simulink model "MMC_Per_arm_outer_v5_G2_case2_clip_delay1p4_aligned"  (R2024a)
settings: Solver=FixedStepDiscrete  StartTime=0.0  StopTime=2  FixedStep=Ts  RelTol=1e-3
PreLoadFcn:
  | % ---- MMC_Inner4 workspace parameters (control gains live inside the MATLAB Function blocks) ----
  | % ---------------- Converter ----------------
  | VDC     = 800;                  % DC-link voltage (V)  -> Vdc_pos / Vdc_neg = VDC/2
  | N       = 8;                    % submodules per arm
  | C       = 2.2e-3;               % submodule capacitance (F)  -> HB_xx blocks
  | vo      = 100;                  % nominal = initial capacitor voltage (V) = VDC/N  -> HB_xx, Vc_nom
  | W_nom   = 0.5*C*N*vo^2;         % nominal arm energy (J) -> initial condition of the Comm delay blocks
  | Larm    = 5e-3;                 % arm inductance (H)
  | Rarm    = 0.5;                  % arm resistance (ohm)
  | 
  | % ---------------- Grid and PCC filter ----------------
  | f       = 50;                   % grid frequency (Hz)
  | Vg_rms  = 230;                  % grid RMS voltage (V)
  | Vg_pk   = Vg_rms*sqrt(2);       % grid peak voltage (V) -> AC Voltage Source
  | Lg      = 2e-3;                 % line inductance (H)
  | Rg      = 0.1;                  % line resistance (ohm)
  | Cf      = 10e-6;                % AC filter capacitance (F)
  | Rf      = 10;                   % AC filter damping resistance (ohm)
  | 
  | % ---------------- Power set-points ----------------
  | Pstar   = 1500;                 % active-power set-point (W)
  | Qstar   = 0;                    % reactive-power set-point (var)
  | 
  | % ---------------- Timing ----------------
  | fsw     = 1250;                 % carrier frequency per submodule (Hz) -> N*fsw = 10 kHz per arm
  | Ts      = 1e-5;                 % simulation step = submodule-layer step (s)
  | Ts_ctrl = 1e-4;                 % arm-leader control step (s)
  | % ---------------- Test schedule: P* staircase and PCC load (added in _tests) ----------------
  | P_base   = 1500;                % staircase base = first level (W)
  | dP_step  = 250;                 % staircase step (W): 1500 -> 1750 -> 2000 -> 2250 -> 2500
  | t_step   = [0.6 1.0 1.4 1.8];   % step instants (s), 0.4 s hold at each level
  | t_back   = 2.2;                 % return to P_base (s) before the load test
  | P_load1  = 1000;                % PCC load 1 (W at 230 V rms)
  | P_load2  = 1000;                % PCC load 2 (W at 230 V rms)
  | R_load1  = Vg_rms^2/P_load1;    % 52.9 ohm
  | R_load2  = Vg_rms^2/P_load2;    % 52.9 ohm
  | t_load1  = 2.4;                 % Breaker load 1: closes at 2.4 s (stays closed)
  | t_load2  = [2.7 3.0];           % Breaker load 2: closes at 2.7 s, opens at 3.0 s
  | % ---- CASE: initial imbalance HB_u3 = 110 V, HB_u6 = 90 V, P* fixed 1500 W, no PCC load, 2 s
  | % ---- DERIVED: case2_clip_delay1p4_aligned: case 2 clip + time-aligned delay 140 samples (1.4 ms) -- eq. (6) test below the bound
  | % ---- DERIVED: case2_clip: same as case 2 + correction bounded to |k_v*err| <= 0.1 in hb_sm_local_ctrl (16 charts)
  | % P_SLEW = 5000 W/s, I_max = 17 A, P_max = 2500 W are set INSIDE mmc_outer_ctrl (both arm leaders)
  | t_load1  = 10;  t_load2 = [10 11];   % PCC load test disabled in this case (beyond StopTime)
  | Vc0_u3   = 110;                 % initial capacitor voltage of HB_u3 (V)
  | Vc0_u6   = 90;                  % initial capacitor voltage of HB_u6 (V)
InitFcn:
  | % ---- MMC_Inner4 workspace parameters (control gains live inside the MATLAB Function blocks) ----
  | % ---------------- Converter ----------------
  | VDC     = 800;                  % DC-link voltage (V)  -> Vdc_pos / Vdc_neg = VDC/2
  | N       = 8;                    % submodules per arm
  | C       = 2.2e-3;               % submodule capacitance (F)  -> HB_xx blocks
  | vo      = 100;                  % nominal = initial capacitor voltage (V) = VDC/N  -> HB_xx, Vc_nom
  | W_nom   = 0.5*C*N*vo^2;         % nominal arm energy (J) -> initial condition of the Comm delay blocks
  | Larm    = 5e-3;                 % arm inductance (H)
  | Rarm    = 0.5;                  % arm resistance (ohm)
  | 
  | % ---------------- Grid and PCC filter ----------------
  | f       = 50;                   % grid frequency (Hz)
  | Vg_rms  = 230;                  % grid RMS voltage (V)
  | Vg_pk   = Vg_rms*sqrt(2);       % grid peak voltage (V) -> AC Voltage Source
  | Lg      = 2e-3;                 % line inductance (H)
  | Rg      = 0.1;                  % line resistance (ohm)
  | Cf      = 10e-6;                % AC filter capacitance (F)
  | Rf      = 10;                   % AC filter damping resistance (ohm)
  | 
  | % ---------------- Power set-points ----------------
  | Pstar   = 1500;                 % active-power set-point (W)
  | Qstar   = 0;                    % reactive-power set-point (var)
  | 
  | % ---------------- Timing ----------------
  | fsw     = 1250;                 % carrier frequency per submodule (Hz) -> N*fsw = 10 kHz per arm
  | Ts      = 1e-5;                 % simulation step = submodule-layer step (s)
  | Ts_ctrl = 1e-4;                 % arm-leader control step (s)
  | % ---------------- Test schedule: P* staircase and PCC load (added in _tests) ----------------
  | P_base   = 1500;                % staircase base = first level (W)
  | dP_step  = 250;                 % staircase step (W): 1500 -> 1750 -> 2000 -> 2250 -> 2500
  | t_step   = [0.6 1.0 1.4 1.8];   % step instants (s), 0.4 s hold at each level
  | t_back   = 2.2;                 % return to P_base (s) before the load test
  | P_load1  = 1000;                % PCC load 1 (W at 230 V rms)
  | P_load2  = 1000;                % PCC load 2 (W at 230 V rms)
  | R_load1  = Vg_rms^2/P_load1;    % 52.9 ohm
  | R_load2  = Vg_rms^2/P_load2;    % 52.9 ohm
  | t_load1  = 2.4;                 % Breaker load 1: closes at 2.4 s (stays closed)
  | t_load2  = [2.7 3.0];           % Breaker load 2: closes at 2.7 s, opens at 3.0 s
  | % ---- CASE: initial imbalance HB_u3 = 110 V, HB_u6 = 90 V, P* fixed 1500 W, no PCC load, 2 s
  | % ---- DERIVED: case2_clip_delay1p4_aligned: case 2 clip + time-aligned delay 140 samples (1.4 ms) -- eq. (6) test below the bound
  | % ---- DERIVED: case2_clip: same as case 2 + correction bounded to |k_v*err| <= 0.1 in hb_sm_local_ctrl (16 charts)
  | % P_SLEW = 5000 W/s, I_max = 17 A, P_max = 2500 W are set INSIDE mmc_outer_ctrl (both arm leaders)
  | t_load1  = 10;  t_load2 = [10 11];   % PCC load test disabled in this case (beyond StopTime)
  | Vc0_u3   = 110;                 % initial capacitor voltage of HB_u3 (V)
  | Vc0_u6   = 90;                  % initial capacitor voltage of HB_u6 (V)
libraries: spsHalfBridgeMMCLib x16, spsSeriesRLCBranchLib x6, spsCurrentMeasurementLib x5, spsBreakerLib x2, spsGroundLib x2, spsDCVoltageSourceLib x2, spsACVoltageSourceLib x1, spspowerguiLib x1, spsVoltageMeasurementLib x1
(part 1 of 6)
settings Model: Creator=Dell  LastModifiedBy=Dell
settings SolverCC: AutoInsertRateTranBlk=on

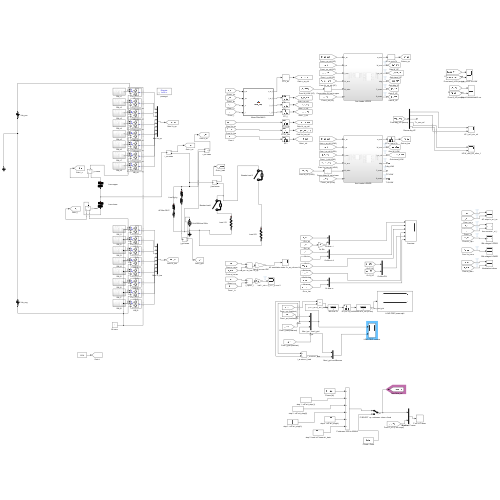
[thumbnail: Simulink's stored preview of the top-level diagram]
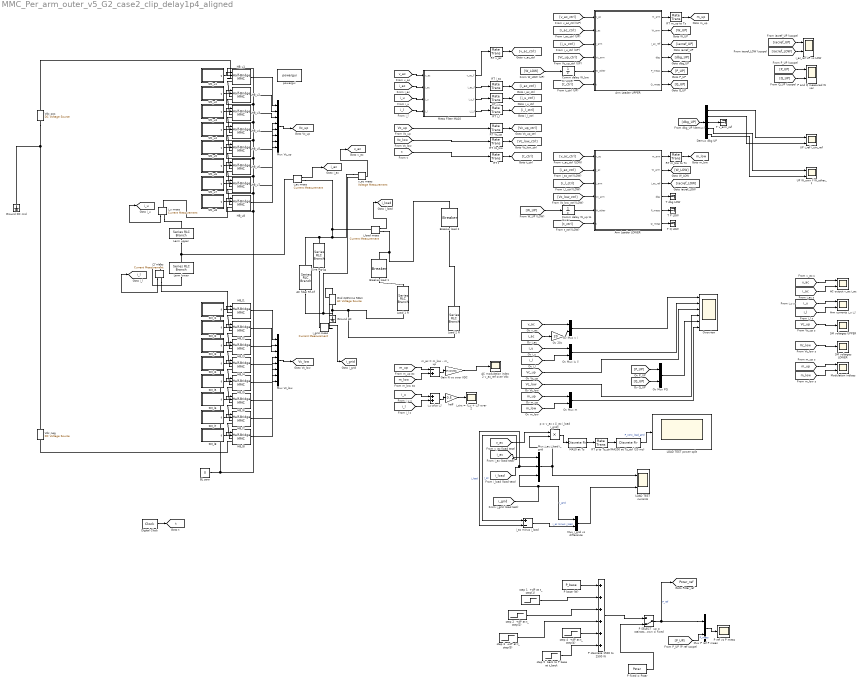
== system MMC_Per_arm_outer_v5_G2_case2_clip_delay1p4_aligned ==
  AC filter Rf-Cf : spsSeriesRLCBranchLib/Series RLC Branch  LConnTagsString=__new0  RConnTagsString=__new0  BranchType=RC  Resistance=Rf  Inductance=1e-3  SetiL0=off  InitialCurrent=0  Capacitance=Cf  Setx0=off  InitialVoltage=0  Measurements=None
  AC modulation index 2 v_ac_ref over Vdc : Scope
  AC output v_ac i_ac : Scope  NumInputPorts=2
  Arm Leader LOWER : Subsystem
  Arm Leader UPPER : Subsystem
  Arm currents i_u i_l : Scope  NumInputPorts=2
  BL zero : Constant  Value=0
  Breaker load 1 : spsBreakerLib/Breaker  InitialState=0  SwitchingTimes=t_load1  External=off  BreakerResistance=0.01  SnubberResistance=1e6  SnubberCapacitance=inf  Measurements=None  MoreParameters=on  NoBreakLoop=off
  Breaker load 2 : spsBreakerLib/Breaker  InitialState=0  SwitchingTimes=t_load2  External=off  BreakerResistance=0.01  SnubberResistance=1e6  SnubberCapacitance=inf  Measurements=None  MoreParameters=on  NoBreakLoop=off
  Comm delay W_low to upper : UnitDelay  InitialCondition=W_nom  SampleTime=Ts_ctrl  HasFrameUpgradeWarning=on
  Comm delay W_up to lower : UnitDelay  InitialCondition=W_nom  SampleTime=Ts_ctrl  HasFrameUpgradeWarning=on
  Demux dbg UP : Demux  Outputs=5
  Digital Clock : DigitalClock  SampleTime=Ts
  Gain N vo over VDC : Gain  Gain=N*vo/VDC
  Grid 230Vrms 50Hz : spsACVoltageSourceLib/AC Voltage Source  Amplitude=Vg_pk  Phase=0  Frequency=f  SampleTime=0  Measurements=None  BusType=swing  Pref=10e3  Qref=0  Qmin=-inf  Qmax=+inf
  Ground AC : spsGroundLib/Ground  LConnTagsString=a
  Ground DC mid : spsGroundLib/Ground  LConnTagsString=a
  HB_l{1..8} (8 alike) : spsHalfBridgeMMCLib/Half-Bridge MMC  ModelType=Switching devices  n=1  C=C  Vc_Initial=vo  Ron=1e-3  Rs=1e6  Cs=inf  Ron_Diode=1e-3  Rs_Diode=1e6  Cs_Diode=inf  Vf_Diode=1e-3  Rs_CurrentSource=inf  Ts=Ts
  HB_u{1..2,4..5,7..8} (6 alike) : spsHalfBridgeMMCLib/Half-Bridge MMC  ModelType=Switching devices  n=1  C=C  Vc_Initial=vo  Ron=1e-3  Rs=1e6  Cs=inf  Ron_Diode=1e-3  Rs_Diode=1e6  Cs_Diode=inf  Vf_Diode=1e-3  Rs_CurrentSource=inf  Ts=Ts
  HB_u3 : spsHalfBridgeMMCLib/Half-Bridge MMC  ModelType=Switching devices  n=1  C=C  Vc_Initial=Vc0_u3  Ron=1e-3  Rs=1e6  Cs=inf  Ron_Diode=1e-3  Rs_Diode=1e6  Cs_Diode=inf  Vf_Diode=1e-3  Rs_CurrentSource=inf  Ts=Ts
  HB_u6 : spsHalfBridgeMMCLib/Half-Bridge MMC  ModelType=Switching devices  n=1  C=C  Vc_Initial=Vc0_u6  Ron=1e-3  Rs=1e6  Cs=inf  Ron_Diode=1e-3  Rs_Diode=1e6  Cs_Diode=inf  Vf_Diode=1e-3  Rs_CurrentSource=inf  Ts=Ts
  LOAD TEST currents : Scope  NumInputPorts=2
  LOAD TEST power split : Scope
  Larm lower : spsSeriesRLCBranchLib/Series RLC Branch  LConnTagsString=__new0  RConnTagsString=__new0  BranchType=RL  Resistance=Rarm  Inductance=Larm  SetiL0=off  InitialCurrent=0  Capacitance=1e-6  Setx0=off  InitialVoltage=0  Measurements=None
  Larm upper : spsSeriesRLCBranchLib/Series RLC Branch  LConnTagsString=__new0  RConnTagsString=__new0  BranchType=RL  Resistance=Rarm  Inductance=Larm  SetiL0=off  InitialCurrent=0  Capacitance=1e-6  Setx0=off  InitialVoltage=0  Measurements=None
  Line Rg-Lg : spsSeriesRLCBranchLib/Series RLC Branch  LConnTagsString=__new0  RConnTagsString=__new0  BranchType=RL  Resistance=Rg  Inductance=Lg  SetiL0=off  InitialCurrent=0  Capacitance=1e-6  Setx0=off  InitialVoltage=0  Measurements=None
  Load 1 R : spsSeriesRLCBranchLib/Series RLC Branch  LConnTagsString=__new0  RConnTagsString=__new0  BranchType=R  Resistance=R_load1  Inductance=1e-3  SetiL0=off  InitialCurrent=0  Capacitance=1e-6  Setx0=off  InitialVoltage=0  Measurements=None
  Load 2 R : spsSeriesRLCBranchLib/Series RLC Branch  LConnTagsString=__new0  RConnTagsString=__new0  BranchType=R  Resistance=R_load2  Inductance=1e-3  SetiL0=off  InitialCurrent=0  Capacitance=1e-6  Setx0=off  InitialVoltage=0  Measurements=None
  MA10 at Ts : DiscreteFir  Coefficients=ones(1,10)/10  SampleTime=Ts
  MA200 at Ts_ctrl (20 ms) : DiscreteFir  Coefficients=ones(1,200)/200  SampleTime=Ts_ctrl
  Meas Filter MA10 : MATLAB Function  TreatAsAtomicUnit=on
  Modulation indices : Scope  NumInputPorts=2
  Mux P ref P meas : Mux  Inputs=2
  Mux Vc_low : Mux  Inputs=8
  Mux Vc_up : Mux  Inputs=8
  Mux i_ac i_load i_grid : Mux  Inputs=3
  Mux i_grid vs difference : Mux  Inputs=2
  Ov 20x : Gain  Gain=20
  Ov Mux PQ : Mux  Inputs=2
  Ov Mux iu il : Mux  Inputs=2
  Ov Mux m : Mux  Inputs=2
  Ov Mux v i : Mux  Inputs=2
  Overview : Scope  NumInputPorts=6
  P SELECT  up = staircase  down = fixed : ManualSwitch  sw=0
  P and Q measured W var : Scope  NumInputPorts=2
  P base (W) : Constant  Value=P_base
  P fixed = Pstar : Constant  Value=Pstar
  P ref vs P meas : Scope
  P staircase 1500 to 2500 W : Sum  Inputs=++++++
  RT Vc_low : RateTransition  OutPortSampleTime=Ts_ctrl
  RT Vc_up : RateTransition  OutPortSampleTime=Ts_ctrl
  RT i_ac : RateTransition  OutPortSampleTime=Ts_ctrl
  RT i_l : RateTransition  OutPortSampleTime=Ts_ctrl
  RT i_u : RateTransition  OutPortSampleTime=Ts_ctrl
  RT m_low to Ts : RateTransition  Deterministic=off  OutPortSampleTime=Ts
  RT m_up to Ts : RateTransition  Deterministic=off  OutPortSampleTime=Ts
  RT p to Ts_ctrl : RateTransition  OutPortSampleTime=Ts_ctrl
  RT t : RateTransition  OutPortSampleTime=Ts_ctrl
  RT v_ac : RateTransition  OutPortSampleTime=Ts_ctrl
  SM voltages LOWER : Scope
  SM voltages UPPER : Scope
  SM_l1 : Subsystem
  SM_l2 : Subsystem
  SM_l3 : Subsystem
  SM_l4 : Subsystem
  SM_l5 : Subsystem
  SM_l6 : Subsystem
  SM_l7 : Subsystem
  SM_l8 : Subsystem
  SM_u1 : Subsystem
  SM_u2 : Subsystem
  SM_u3 : Subsystem
  SM_u4 : Subsystem
  SM_u5 : Subsystem
  SM_u6 : Subsystem
  SM_u7 : Subsystem
  SM_u8 : Subsystem
  T P LOW : Terminator
  T Q LOW : Terminator
  T dbg LOW : Terminator
  T v_arm_ref : Terminator
  UP W_own_f W_other_f : Scope  NumInputPorts=2
  UP i_ref i_circ_ref : Scope  NumInputPorts=2
  Vdc_neg : spsDCVoltageSourceLib/DC Voltage Source  Amplitude=VDC/2  Measurements=None
  Vdc_pos : spsDCVoltageSourceLib/DC Voltage Source  Amplitude=VDC/2  Measurements=None
  half : Gain  Gain=0.5
  i_ac meas : spsCurrentMeasurementLib/Current Measurement  PhasorSimulation=off  OutputType=Complex  PSBequivalent=0
  i_ac minus i_load : Sum  Inputs=+-
  i_ac_ref UP vs LOW : Scope  NumInputPorts=2
  i_circ = (i_u + i_l) over 2 : Scope
  i_grid meas : spsCurrentMeasurementLib/Current Measurement  PhasorSimulation=off  OutputType=Complex  PSBequivalent=0
  i_l meas : spsCurrentMeasurementLib/Current Measurement  PhasorSimulation=off  OutputType=Complex  PSBequivalent=0
  i_load meas : spsCurrentMeasurementLib/Current Measurement  PhasorSimulation=off  OutputType=Complex  PSBequivalent=0
  i_u meas : spsCurrentMeasurementLib/Current Measurement  PhasorSimulation=off  OutputType=Complex  PSBequivalent=0
  i_u plus i_l : Sum
  m_ac = m_low - m_up : Sum  Inputs=-+
  p = v_ac x [i_ac i_load i_grid] : Product
  powergui : spspowerguiLib/powergui  Priority=1  SimulationMode=Discrete  SampleTime=Ts  frequency=50  Iterations=50  frequencyindice=50  Pbase=100e6  ErrMax=1e-4  UnitsV=kV  UnitsW=MW  buscounter=0  FunctionMessages=off  echomessages=off  EnableUseOfTLC=off  CurrentSourceSwitches=off  DisableSnubberDevices=off  DisableRonSwitches=off  DisableVfSwitches=off  DisplayEquations=off  AutomaticDiscreteSolvers=off  SolverType=Tustin/Backward Euler (TBE)  Interpol=off  ExternalGateDelay=off  methode=off  Ts=100  x0status=blocks  SPID=on  SwTol=0  HookPort=off  NonlinearTolerance=1e-4  nMaxIteration=100  ContinueOnMaxIteration=off  RestoreLinks=warning  ResistiveCurrentMeasurement=off  Frange=[0:2:500]  Ylog=off  Xlog=on  ShowGrid=off  save=off  variable=ZData  structure=0  ZoomFFT=off  StartTime=0.0  cycles=1  DisplayStyle=1  fundamental=50  FreqAxis=off  MaxFrequency=1000  frequencyindicesteady=1  RmsSteady=1  display=off
  step 1  +dP at t_step(1) : Step  Time=t_step(1)  After=dP_step  SampleTime=Ts_ctrl
  step 2  +dP at t_step(2) : Step  Time=t_step(2)  After=dP_step  SampleTime=Ts_ctrl
  step 3  +dP at t_step(3) : Step  Time=t_step(3)  After=dP_step  SampleTime=Ts_ctrl
  step 4  +dP at t_step(4) : Step  Time=t_step(4)  After=dP_step  SampleTime=Ts_ctrl
  step 5  back to P base at t_back : Step  Time=t_back  After=-4*dP_step  SampleTime=Ts_ctrl
  v_ac meas : spsVoltageMeasurementLib/Voltage Measurement  PhasorSimulation=off  OutputType=Complex  PSBequivalent=0
  tag scope: Pstar_ref=global, Vc_low=global, Vc_up=global, i_ac=global, i_grid=global, i_l=global, i_load=global, i_u=global, m_low=global, m_up=global, t=global, v_ac=global
  wires:
  v_ac meas/1 -> [v_ac]
  i_ac meas/1 -> [i_ac]
  i_u meas/1 -> [i_u]
  i_l meas/1 -> [i_l]
  BL zero/1 -> HB_u1/2, HB_u2/2, HB_u3/2, HB_u4/2, HB_u5/2, HB_u6/2, HB_u7/2, HB_u8/2, HB_l1/2, HB_l2/2, HB_l3/2, HB_l4/2, HB_l5/2, HB_l6/2, HB_l7/2, HB_l8/2
  HB_u1/1 -> Mux Vc_up/1
  HB_l1/1 -> Mux Vc_low/1
  HB_u2/1 -> Mux Vc_up/2
  HB_l2/1 -> Mux Vc_low/2
  HB_u3/1 -> Mux Vc_up/3
  HB_l3/1 -> Mux Vc_low/3
  HB_u4/1 -> Mux Vc_up/4
  HB_l4/1 -> Mux Vc_low/4
  HB_u5/1 -> Mux Vc_up/5
  HB_l5/1 -> Mux Vc_low/5
  HB_u6/1 -> Mux Vc_up/6
  HB_l6/1 -> Mux Vc_low/6
  HB_u7/1 -> Mux Vc_up/7
  HB_l7/1 -> Mux Vc_low/7
  HB_u8/1 -> Mux Vc_up/8
  HB_l8/1 -> Mux Vc_low/8
  Mux Vc_up/1 -> [Vc_up]
  Mux Vc_low/1 -> [Vc_low]
  Digital Clock/1 -> [t]
  SM_u1/1(g) -> HB_u1/1
  SM_l1/1(g) -> HB_l1/1
  SM_u2/1(g) -> HB_u2/1
  SM_l2/1(g) -> HB_l2/1
  SM_u3/1(g) -> HB_u3/1
  SM_l3/1(g) -> HB_l3/1
  SM_u4/1(g) -> HB_u4/1
  SM_l4/1(g) -> HB_l4/1
  SM_u5/1(g) -> HB_u5/1
  SM_l5/1(g) -> HB_l5/1
  SM_u6/1(g) -> HB_u6/1
  SM_l6/1(g) -> HB_l6/1
  SM_u7/1(g) -> HB_u7/1
  SM_l7/1(g) -> HB_l7/1
  SM_u8/1(g) -> HB_u8/1
  SM_l8/1(g) -> HB_l8/1
  [v_ac] -> Meas Filter MA10/1(v_ac)
  [i_ac] -> Meas Filter MA10/2(i_ac)
  [i_u] -> Meas Filter MA10/3(i_u)
  [i_l] -> Meas Filter MA10/4(i_l)
  Meas Filter MA10/1(v_ac_f) -> RT v_ac/1
  Meas Filter MA10/2(i_ac_f) -> RT i_ac/1
  Meas Filter MA10/3(i_u_f) -> RT i_u/1
  Meas Filter MA10/4(i_l_f) -> RT i_l/1
  [Vc_up] -> RT Vc_up/1
  [Vc_low] -> RT Vc_low/1
  [t] -> RT t/1
  [v_ac] -> AC output v_ac i_ac/1
  [i_ac] -> AC output v_ac i_ac/2
  [i_u] -> Arm currents i_u i_l/1
  [i_l] -> Arm currents i_u i_l/2
  [Vc_up] -> SM voltages UPPER/1
  [Vc_low] -> SM voltages LOWER/1
  [m_up] -> Modulation indices/1
  [m_low] -> Modulation indices/2
  [m_up] -> m_ac = m_low - m_up/1
  [m_low] -> m_ac = m_low - m_up/2
  m_ac = m_low - m_up/1 -> Gain N vo over VDC/1
  Gain N vo over VDC/1 -> AC modulation index 2 v_ac_ref over Vdc/1
  [i_u] -> i_u plus i_l/1
  [i_l] -> i_u plus i_l/2
  i_u plus i_l/1 -> half/1
  half/1 -> i_circ = (i_u + i_l) over 2/1
  Demux dbg UP/1 -> UP i_ref i_circ_ref/1
  Demux dbg UP/2 -> UP i_ref i_circ_ref/2
  Demux dbg UP/3 -> T v_arm_ref/1
  Demux dbg UP/4 -> UP W_own_f W_other_f/1
  Demux dbg UP/5 -> UP W_own_f W_other_f/2
  [v_ac] -> Ov Mux v i/1
  [i_ac] -> Ov 20x/1
  Ov 20x/1 -> Ov Mux v i/2
  [i_u] -> Ov Mux iu il/1
  [i_l] -> Ov Mux iu il/2
  [m_up] -> Ov Mux m/1
  [m_low] -> Ov Mux m/2
  Ov Mux v i/1 -> Overview/1
  Ov Mux iu il/1 -> Overview/2
  [Vc_up] -> Overview/3
  [Vc_low] -> Overview/4
  Ov Mux PQ/1 -> Overview/5
  Ov Mux m/1 -> Overview/6
  RT v_ac/1 -> [v_ac_ctrl]
  RT i_ac/1 -> [i_ac_ctrl]
  RT i_u/1 -> [i_u_ctrl]
  RT i_l/1 -> [i_l_ctrl]
  RT Vc_up/1 -> [Vc_up_ctrl]
  RT Vc_low/1 -> [Vc_low_ctrl]
  RT t/1 -> [t_ctrl]
  [v_ac_ctrl] -> Arm Leader UPPER/1(v_ac)
  [i_ac_ctrl] -> Arm Leader UPPER/2(i_ac)
  [i_u_ctrl] -> Arm Leader UPPER/3(i_arm)
  [Vc_up_ctrl] -> Arm Leader UPPER/4(Vc_arm)
  [W_LOW] -> Comm delay W_low to upper/1
  Comm delay W_low to upper/1 -> Arm Leader UPPER/5(W_other)
  [t_ctrl] -> Arm Leader UPPER/6(t)
  [v_ac_ctrl] -> Arm Leader LOWER/1(v_ac)
  [i_ac_ctrl] -> Arm Leader LOWER/2(i_ac)
  [i_l_ctrl] -> Arm Leader LOWER/3(i_arm)
  [Vc_low_ctrl] -> Arm Leader LOWER/4(Vc_arm)
  [W_UP] -> Comm delay W_up to lower/1
  Comm delay W_up to lower/1 -> Arm Leader LOWER/5(W_other)
  [t_ctrl] -> Arm Leader LOWER/6(t)
  Arm Leader UPPER/1(m_arm) -> RT m_up to Ts/1
  RT m_up to Ts/1 -> [m_up]
  Arm Leader UPPER/2(W_arm) -> [W_UP]
  Arm Leader UPPER/3(i_ac_ref) -> [iacref_UP]
  Arm Leader UPPER/4(dbg) -> [dbg_UP]
  Arm Leader UPPER/5(P_meas) -> [P_UP]
  Arm Leader UPPER/6(Q_meas) -> [Q_UP]
  Arm Leader LOWER/1(m_arm) -> RT m_low to Ts/1
  RT m_low to Ts/1 -> [m_low]
  Arm Leader LOWER/2(W_arm) -> [W_LOW]
  Arm Leader LOWER/3(i_ac_ref) -> [iacref_LOW]
  Arm Leader LOWER/4(dbg) -> T dbg LOW/1
  Arm Leader LOWER/5(P_meas) -> T P LOW/1
  Arm Leader LOWER/6(Q_meas) -> T Q LOW/1
  [iacref_UP] -> i_ac_ref UP vs LOW/1
  [iacref_LOW] -> i_ac_ref UP vs LOW/2
  [P_UP] -> P and Q measured W var/1
  [Q_UP] -> P and Q measured W var/2
  [dbg_UP] -> Demux dbg UP/1
  [P_UP] -> Ov Mux PQ/1
  [Q_UP] -> Ov Mux PQ/2
  P base (W)/1 -> P staircase 1500 to 2500 W/1
  step 1  +dP at t_step(1)/1 -> P staircase 1500 to 2500 W/2
  step 2  +dP at t_step(2)/1 -> P staircase 1500 to 2500 W/3
  step 3  +dP at t_step(3)/1 -> P staircase 1500 to 2500 W/4
  step 4  +dP at t_step(4)/1 -> P staircase 1500 to 2500 W/5
  step 5  back to P base at t_back/1 -> P staircase 1500 to 2500 W/6
  P staircase 1500 to 2500 W/1 -> P SELECT  up = staircase  down = fixed/1
  P fixed = Pstar/1 -> P SELECT  up = staircase  down = fixed/2
  P SELECT  up = staircase  down = fixed/1 -> [Pstar_ref], Mux P ref P meas/1  "P_ref"
  [P_UP] -> Mux P ref P meas/2  "P_meas"
  Mux P ref P meas/1 -> P ref vs P meas/1
  i_load meas/1 -> [i_load]
  i_grid meas/1 -> [i_grid]
  [i_ac] -> Mux i_ac i_load i_grid/1, i_ac minus i_load/1  "i_ac"
  [i_load] -> Mux i_ac i_load i_grid/2, i_ac minus i_load/2  "i_load"
  [i_grid] -> Mux i_ac i_load i_grid/3, Mux i_grid vs difference/1  "i_grid"
  i_ac minus i_load/1 -> Mux i_grid vs difference/2  "i_ac minus i_load"
  Mux i_ac i_load i_grid/1 -> p = v_ac x [i_ac i_load i_grid]/2, LOAD TEST currents/1
  Mux i_grid vs difference/1 -> LOAD TEST currents/2
  [v_ac] -> p = v_ac x [i_ac i_load i_grid]/1
  p = v_ac x [i_ac i_load i_grid]/1 -> MA10 at Ts/1
  MA10 at Ts/1 -> RT p to Ts_ctrl/1
  RT p to Ts_ctrl/1 -> MA200 at Ts_ctrl (20 ms)/1
  MA200 at Ts_ctrl (20 ms)/1 -> LOAD TEST power split/1  "P_conv_load_grid"
  connections:
  HB_u1/LConn1 -- Vdc_pos/RConn1
  Vdc_pos/LConn1 -- Ground DC mid/LConn1 -- Vdc_neg/RConn1
  HB_u1/LConn2 -- HB_u2/LConn1
  HB_l1/LConn2 -- HB_l2/LConn1
  HB_u2/LConn2 -- HB_u3/LConn1
  HB_l2/LConn2 -- HB_l3/LConn1
  HB_u3/LConn2 -- HB_u4/LConn1
  HB_l3/LConn2 -- HB_l4/LConn1
  HB_u4/LConn2 -- HB_u5/LConn1
  HB_l4/LConn2 -- HB_l5/LConn1
  HB_u5/LConn2 -- HB_u6/LConn1
  HB_l5/LConn2 -- HB_l6/LConn1
  HB_u6/LConn2 -- HB_u7/LConn1
  HB_l6/LConn2 -- HB_l7/LConn1
  HB_u7/LConn2 -- HB_u8/LConn1
  HB_l7/LConn2 -- HB_l8/LConn1
  HB_u8/LConn2 -- i_u meas/LConn1
  i_u meas/RConn1 -- Larm upper/LConn1
  Larm upper/RConn1 -- i_ac meas/LConn1 -- Larm lower/LConn1
  Larm lower/RConn1 -- i_l meas/LConn1
  i_l meas/RConn1 -- HB_l1/LConn1
  HB_l8/LConn2 -- Vdc_neg/LConn1
  v_ac meas/LConn1 -- Line Rg-Lg/LConn1 -- AC filter Rf-Cf/LConn1 -- i_ac meas/RConn1 -- i_load meas/LConn1
  Line Rg-Lg/RConn1 -- i_grid meas/LConn1
  Grid 230Vrms 50Hz/LConn1 -- Load 1 R/RConn1 -- Load 2 R/RConn1 -- AC filter Rf-Cf/RConn1 -- v_ac meas/LConn2 -- Ground AC/LConn1
  i_load meas/RConn1 -- Breaker load 2/LConn1 -- Breaker load 1/LConn1
  Breaker load 1/RConn1 -- Load 1 R/LConn1
  Breaker load 2/RConn1 -- Load 2 R/LConn1
  i_grid meas/RConn1 -- Grid 230Vrms 50Hz/RConn1

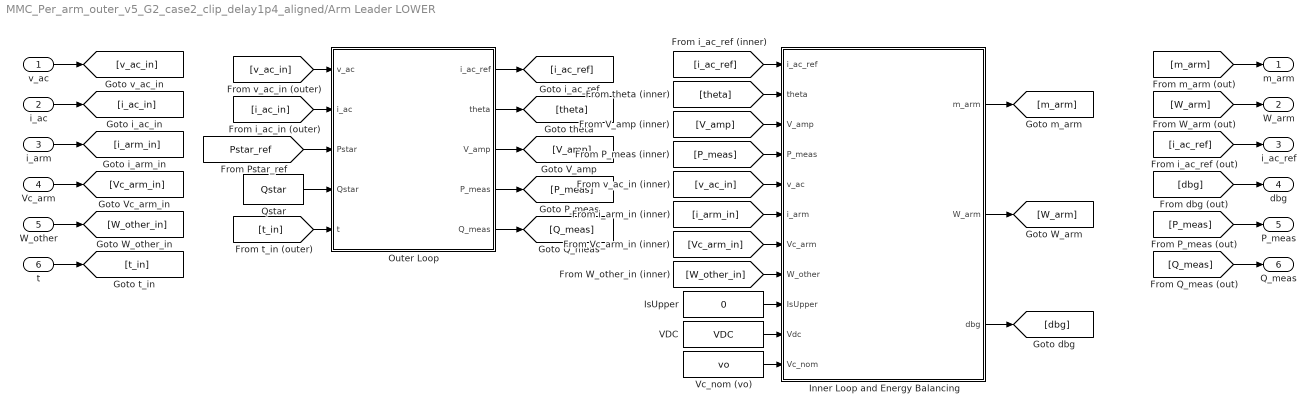
== system MMC_Per_arm_outer_v5_G2_case2_clip_delay1p4_aligned/Arm Leader LOWER ==
  v_ac : Inport
  i_ac : Inport  Port=2
  i_arm : Inport  Port=3
  Vc_arm : Inport  Port=4
  W_other : Inport  Port=5
  t : Inport  Port=6
  Inner Loop and Energy Balancing : Subsystem
  IsUpper : Constant  Value=0
  Outer Loop : MATLAB Function  TreatAsAtomicUnit=on
  Qstar : Constant  Value=Qstar
  VDC : Constant  Value=VDC
  Vc_nom (vo) : Constant  Value=vo
  m_arm : Outport
  W_arm : Outport  Port=2
  i_ac_ref : Outport  Port=3
  dbg : Outport  Port=4
  P_meas : Outport  Port=5
  Q_meas : Outport  Port=6
  wires:
  v_ac/1 -> [v_ac_in]
  i_ac/1 -> [i_ac_in]
  i_arm/1 -> [i_arm_in]
  Vc_arm/1 -> [Vc_arm_in]
  W_other/1 -> [W_other_in]
  t/1 -> [t_in]
  [v_ac_in] -> Outer Loop/1(v_ac)
  [i_ac_in] -> Outer Loop/2(i_ac)
  [Pstar_ref] -> Outer Loop/3(Pstar)
  Qstar/1 -> Outer Loop/4(Qstar)
  [t_in] -> Outer Loop/5(t)
  Outer Loop/1(i_ac_ref) -> [i_ac_ref]
  Outer Loop/2(theta) -> [theta]
  Outer Loop/3(V_amp) -> [V_amp]
  Outer Loop/4(P_meas) -> [P_meas]
  Outer Loop/5(Q_meas) -> [Q_meas]
  [i_ac_ref] -> Inner Loop and Energy Balancing/1(i_ac_ref)
  [theta] -> Inner Loop and Energy Balancing/2(theta)
  [V_amp] -> Inner Loop and Energy Balancing/3(V_amp)
  [P_meas] -> Inner Loop and Energy Balancing/4(P_meas)
  [v_ac_in] -> Inner Loop and Energy Balancing/5(v_ac)
  [i_arm_in] -> Inner Loop and Energy Balancing/6(i_arm)
  [Vc_arm_in] -> Inner Loop and Energy Balancing/7(Vc_arm)
  [W_other_in] -> Inner Loop and Energy Balancing/8(W_other)
  IsUpper/1 -> Inner Loop and Energy Balancing/9(IsUpper)
  VDC/1 -> Inner Loop and Energy Balancing/10(Vdc)
  Vc_nom (vo)/1 -> Inner Loop and Energy Balancing/11(Vc_nom)
  Inner Loop and Energy Balancing/1(m_arm) -> [m_arm]
  Inner Loop and Energy Balancing/2(W_arm) -> [W_arm]
  Inner Loop and Energy Balancing/3(dbg) -> [dbg]
  [m_arm] -> m_arm/1
  [W_arm] -> W_arm/1
  [i_ac_ref] -> i_ac_ref/1
  [dbg] -> dbg/1
  [P_meas] -> P_meas/1
  [Q_meas] -> Q_meas/1

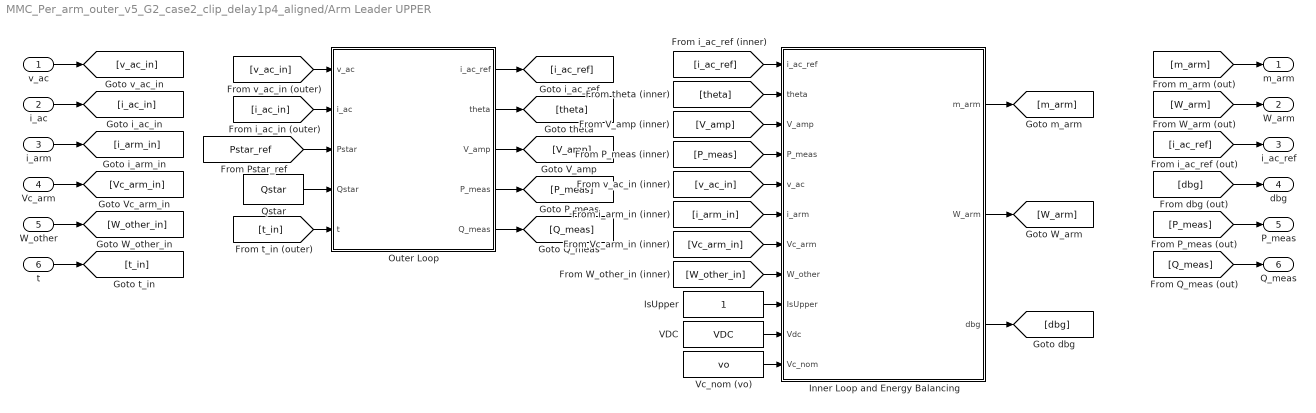
== system MMC_Per_arm_outer_v5_G2_case2_clip_delay1p4_aligned/Arm Leader UPPER ==
  v_ac : Inport
  i_ac : Inport  Port=2
  i_arm : Inport  Port=3
  Vc_arm : Inport  Port=4
  W_other : Inport  Port=5
  t : Inport  Port=6
  Inner Loop and Energy Balancing : Subsystem
  IsUpper : Constant
  Outer Loop : MATLAB Function  TreatAsAtomicUnit=on
  Qstar : Constant  Value=Qstar
  VDC : Constant  Value=VDC
  Vc_nom (vo) : Constant  Value=vo
  m_arm : Outport
  W_arm : Outport  Port=2
  i_ac_ref : Outport  Port=3
  dbg : Outport  Port=4
  P_meas : Outport  Port=5
  Q_meas : Outport  Port=6
  wires:
  v_ac/1 -> [v_ac_in]
  i_ac/1 -> [i_ac_in]
  i_arm/1 -> [i_arm_in]
  Vc_arm/1 -> [Vc_arm_in]
  W_other/1 -> [W_other_in]
  t/1 -> [t_in]
  [v_ac_in] -> Outer Loop/1(v_ac)
  [i_ac_in] -> Outer Loop/2(i_ac)
  [Pstar_ref] -> Outer Loop/3(Pstar)
  Qstar/1 -> Outer Loop/4(Qstar)
  [t_in] -> Outer Loop/5(t)
  Outer Loop/1(i_ac_ref) -> [i_ac_ref]
  Outer Loop/2(theta) -> [theta]
  Outer Loop/3(V_amp) -> [V_amp]
  Outer Loop/4(P_meas) -> [P_meas]
  Outer Loop/5(Q_meas) -> [Q_meas]
  [i_ac_ref] -> Inner Loop and Energy Balancing/1(i_ac_ref)
  [theta] -> Inner Loop and Energy Balancing/2(theta)
  [V_amp] -> Inner Loop and Energy Balancing/3(V_amp)
  [P_meas] -> Inner Loop and Energy Balancing/4(P_meas)
  [v_ac_in] -> Inner Loop and Energy Balancing/5(v_ac)
  [i_arm_in] -> Inner Loop and Energy Balancing/6(i_arm)
  [Vc_arm_in] -> Inner Loop and Energy Balancing/7(Vc_arm)
  [W_other_in] -> Inner Loop and Energy Balancing/8(W_other)
  IsUpper/1 -> Inner Loop and Energy Balancing/9(IsUpper)
  VDC/1 -> Inner Loop and Energy Balancing/10(Vdc)
  Vc_nom (vo)/1 -> Inner Loop and Energy Balancing/11(Vc_nom)
  Inner Loop and Energy Balancing/1(m_arm) -> [m_arm]
  Inner Loop and Energy Balancing/2(W_arm) -> [W_arm]
  Inner Loop and Energy Balancing/3(dbg) -> [dbg]
  [m_arm] -> m_arm/1
  [W_arm] -> W_arm/1
  [i_ac_ref] -> i_ac_ref/1
  [dbg] -> dbg/1
  [P_meas] -> P_meas/1
  [Q_meas] -> Q_meas/1

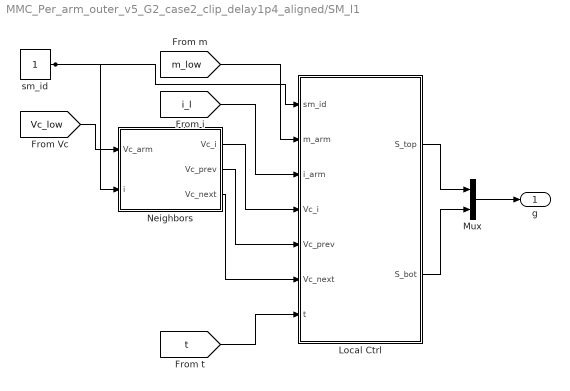
== system MMC_Per_arm_outer_v5_G2_case2_clip_delay1p4_aligned/SM_l1 ==
  Local Ctrl : MATLAB Function  TreatAsAtomicUnit=on
  Mux : Mux  Inputs=2
  Neighbors : MATLAB Function  TreatAsAtomicUnit=on
  sm_id : Constant
  g : Outport
  wires:
  [Vc_low] -> Neighbors/1(Vc_arm)
  sm_id/1 -> Neighbors/2(i), Local Ctrl/1(sm_id)
  [m_low] -> Local Ctrl/2(m_arm)
  [i_l] -> Local Ctrl/3(i_arm)
  Neighbors/1(Vc_i) -> Local Ctrl/4(Vc_i)
  Neighbors/2(Vc_prev) -> Local Ctrl/5(Vc_prev)
  Neighbors/3(Vc_next) -> Local Ctrl/6(Vc_next)
  [t] -> Local Ctrl/7(t)
  Local Ctrl/1(S_top) -> Mux/1
  Local Ctrl/2(S_bot) -> Mux/2
  Mux/1 -> g/1

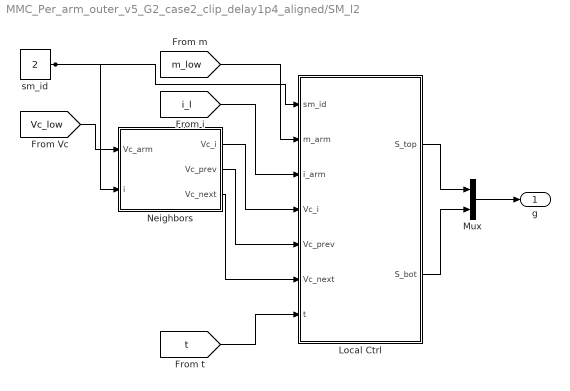
== system MMC_Per_arm_outer_v5_G2_case2_clip_delay1p4_aligned/SM_l2 ==
  Local Ctrl : MATLAB Function  TreatAsAtomicUnit=on
  Mux : Mux  Inputs=2
  Neighbors : MATLAB Function  TreatAsAtomicUnit=on
  sm_id : Constant  Value=2
  g : Outport
  wires:
  [Vc_low] -> Neighbors/1(Vc_arm)
  sm_id/1 -> Neighbors/2(i), Local Ctrl/1(sm_id)
  [m_low] -> Local Ctrl/2(m_arm)
  [i_l] -> Local Ctrl/3(i_arm)
  Neighbors/1(Vc_i) -> Local Ctrl/4(Vc_i)
  Neighbors/2(Vc_prev) -> Local Ctrl/5(Vc_prev)
  Neighbors/3(Vc_next) -> Local Ctrl/6(Vc_next)
  [t] -> Local Ctrl/7(t)
  Local Ctrl/1(S_top) -> Mux/1
  Local Ctrl/2(S_bot) -> Mux/2
  Mux/1 -> g/1

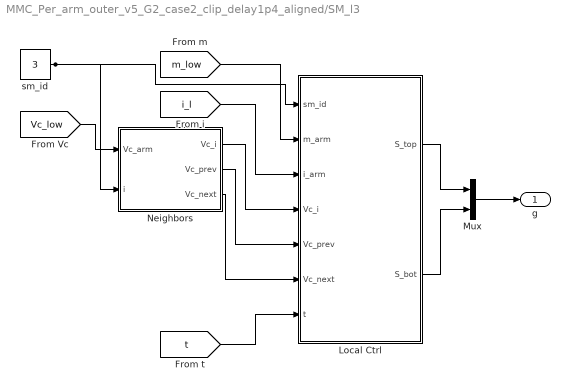
== system MMC_Per_arm_outer_v5_G2_case2_clip_delay1p4_aligned/SM_l3 ==
  Local Ctrl : MATLAB Function  TreatAsAtomicUnit=on
  Mux : Mux  Inputs=2
  Neighbors : MATLAB Function  TreatAsAtomicUnit=on
  sm_id : Constant  Value=3
  g : Outport
  wires:
  [Vc_low] -> Neighbors/1(Vc_arm)
  sm_id/1 -> Neighbors/2(i), Local Ctrl/1(sm_id)
  [m_low] -> Local Ctrl/2(m_arm)
  [i_l] -> Local Ctrl/3(i_arm)
  Neighbors/1(Vc_i) -> Local Ctrl/4(Vc_i)
  Neighbors/2(Vc_prev) -> Local Ctrl/5(Vc_prev)
  Neighbors/3(Vc_next) -> Local Ctrl/6(Vc_next)
  [t] -> Local Ctrl/7(t)
  Local Ctrl/1(S_top) -> Mux/1
  Local Ctrl/2(S_bot) -> Mux/2
  Mux/1 -> g/1

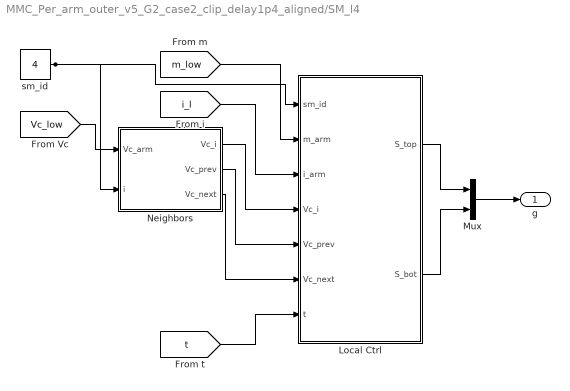
== system MMC_Per_arm_outer_v5_G2_case2_clip_delay1p4_aligned/SM_l4 ==
  Local Ctrl : MATLAB Function  TreatAsAtomicUnit=on
  Mux : Mux  Inputs=2
  Neighbors : MATLAB Function  TreatAsAtomicUnit=on
  sm_id : Constant  Value=4
  g : Outport
  wires:
  [Vc_low] -> Neighbors/1(Vc_arm)
  sm_id/1 -> Neighbors/2(i), Local Ctrl/1(sm_id)
  [m_low] -> Local Ctrl/2(m_arm)
  [i_l] -> Local Ctrl/3(i_arm)
  Neighbors/1(Vc_i) -> Local Ctrl/4(Vc_i)
  Neighbors/2(Vc_prev) -> Local Ctrl/5(Vc_prev)
  Neighbors/3(Vc_next) -> Local Ctrl/6(Vc_next)
  [t] -> Local Ctrl/7(t)
  Local Ctrl/1(S_top) -> Mux/1
  Local Ctrl/2(S_bot) -> Mux/2
  Mux/1 -> g/1

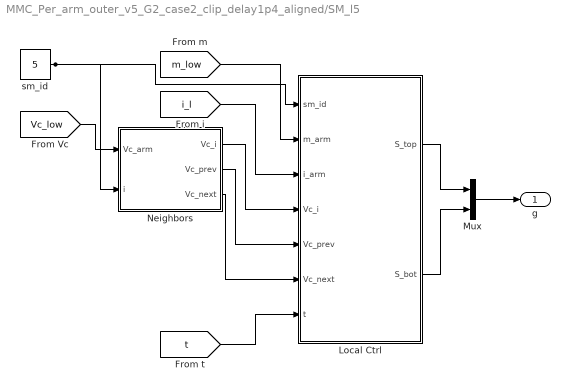
== system MMC_Per_arm_outer_v5_G2_case2_clip_delay1p4_aligned/SM_l5 ==
  Local Ctrl : MATLAB Function  TreatAsAtomicUnit=on
  Mux : Mux  Inputs=2
  Neighbors : MATLAB Function  TreatAsAtomicUnit=on
  sm_id : Constant  Value=5
  g : Outport
  wires:
  [Vc_low] -> Neighbors/1(Vc_arm)
  sm_id/1 -> Neighbors/2(i), Local Ctrl/1(sm_id)
  [m_low] -> Local Ctrl/2(m_arm)
  [i_l] -> Local Ctrl/3(i_arm)
  Neighbors/1(Vc_i) -> Local Ctrl/4(Vc_i)
  Neighbors/2(Vc_prev) -> Local Ctrl/5(Vc_prev)
  Neighbors/3(Vc_next) -> Local Ctrl/6(Vc_next)
  [t] -> Local Ctrl/7(t)
  Local Ctrl/1(S_top) -> Mux/1
  Local Ctrl/2(S_bot) -> Mux/2
  Mux/1 -> g/1

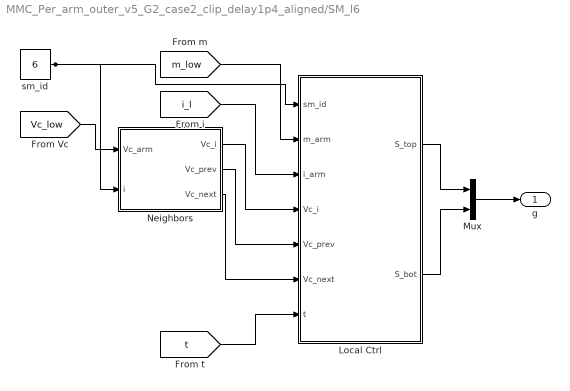
== system MMC_Per_arm_outer_v5_G2_case2_clip_delay1p4_aligned/SM_l6 ==
  Local Ctrl : MATLAB Function  TreatAsAtomicUnit=on
  Mux : Mux  Inputs=2
  Neighbors : MATLAB Function  TreatAsAtomicUnit=on
  sm_id : Constant  Value=6
  g : Outport
  wires:
  [Vc_low] -> Neighbors/1(Vc_arm)
  sm_id/1 -> Neighbors/2(i), Local Ctrl/1(sm_id)
  [m_low] -> Local Ctrl/2(m_arm)
  [i_l] -> Local Ctrl/3(i_arm)
  Neighbors/1(Vc_i) -> Local Ctrl/4(Vc_i)
  Neighbors/2(Vc_prev) -> Local Ctrl/5(Vc_prev)
  Neighbors/3(Vc_next) -> Local Ctrl/6(Vc_next)
  [t] -> Local Ctrl/7(t)
  Local Ctrl/1(S_top) -> Mux/1
  Local Ctrl/2(S_bot) -> Mux/2
  Mux/1 -> g/1

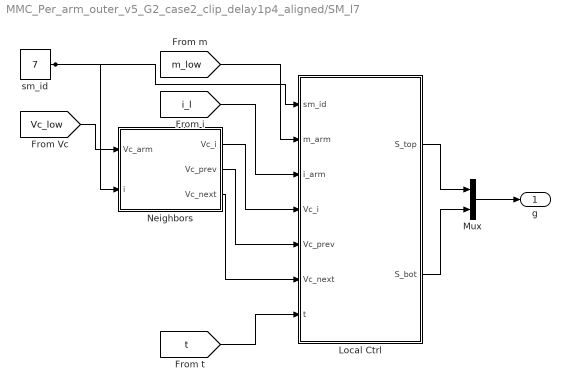
== system MMC_Per_arm_outer_v5_G2_case2_clip_delay1p4_aligned/SM_l7 ==
  Local Ctrl : MATLAB Function  TreatAsAtomicUnit=on
  Mux : Mux  Inputs=2
  Neighbors : MATLAB Function  TreatAsAtomicUnit=on
  sm_id : Constant  Value=7
  g : Outport
  wires:
  [Vc_low] -> Neighbors/1(Vc_arm)
  sm_id/1 -> Neighbors/2(i), Local Ctrl/1(sm_id)
  [m_low] -> Local Ctrl/2(m_arm)
  [i_l] -> Local Ctrl/3(i_arm)
  Neighbors/1(Vc_i) -> Local Ctrl/4(Vc_i)
  Neighbors/2(Vc_prev) -> Local Ctrl/5(Vc_prev)
  Neighbors/3(Vc_next) -> Local Ctrl/6(Vc_next)
  [t] -> Local Ctrl/7(t)
  Local Ctrl/1(S_top) -> Mux/1
  Local Ctrl/2(S_bot) -> Mux/2
  Mux/1 -> g/1

== system MMC_Per_arm_outer_v5_G2_case2_clip_delay1p4_aligned/SM_l8 ==
  Local Ctrl : MATLAB Function  TreatAsAtomicUnit=on
  Mux : Mux  Inputs=2
  Neighbors : MATLAB Function  TreatAsAtomicUnit=on
  sm_id : Constant  Value=8
  g : Outport
  wires:
  [Vc_low] -> Neighbors/1(Vc_arm)
  sm_id/1 -> Neighbors/2(i), Local Ctrl/1(sm_id)
  [m_low] -> Local Ctrl/2(m_arm)
  [i_l] -> Local Ctrl/3(i_arm)
  Neighbors/1(Vc_i) -> Local Ctrl/4(Vc_i)
  Neighbors/2(Vc_prev) -> Local Ctrl/5(Vc_prev)
  Neighbors/3(Vc_next) -> Local Ctrl/6(Vc_next)
  [t] -> Local Ctrl/7(t)
  Local Ctrl/1(S_top) -> Mux/1
  Local Ctrl/2(S_bot) -> Mux/2
  Mux/1 -> g/1

== system MMC_Per_arm_outer_v5_G2_case2_clip_delay1p4_aligned/SM_u1 ==
  Local Ctrl : MATLAB Function  TreatAsAtomicUnit=on
  Mux : Mux  Inputs=2
  Neighbors : MATLAB Function  TreatAsAtomicUnit=on
  sm_id : Constant
  g : Outport
  wires:
  [Vc_up] -> Neighbors/1(Vc_arm)
  sm_id/1 -> Neighbors/2(i), Local Ctrl/1(sm_id)
  [m_up] -> Local Ctrl/2(m_arm)
  [i_u] -> Local Ctrl/3(i_arm)
  Neighbors/1(Vc_i) -> Local Ctrl/4(Vc_i)
  Neighbors/2(Vc_prev) -> Local Ctrl/5(Vc_prev)
  Neighbors/3(Vc_next) -> Local Ctrl/6(Vc_next)
  [t] -> Local Ctrl/7(t)
  Local Ctrl/1(S_top) -> Mux/1
  Local Ctrl/2(S_bot) -> Mux/2
  Mux/1 -> g/1

== system MMC_Per_arm_outer_v5_G2_case2_clip_delay1p4_aligned/SM_u2 ==
  Local Ctrl : MATLAB Function  TreatAsAtomicUnit=on
  Mux : Mux  Inputs=2
  Neighbors : MATLAB Function  TreatAsAtomicUnit=on
  sm_id : Constant  Value=2
  g : Outport
  wires:
  [Vc_up] -> Neighbors/1(Vc_arm)
  sm_id/1 -> Neighbors/2(i), Local Ctrl/1(sm_id)
  [m_up] -> Local Ctrl/2(m_arm)
  [i_u] -> Local Ctrl/3(i_arm)
  Neighbors/1(Vc_i) -> Local Ctrl/4(Vc_i)
  Neighbors/2(Vc_prev) -> Local Ctrl/5(Vc_prev)
  Neighbors/3(Vc_next) -> Local Ctrl/6(Vc_next)
  [t] -> Local Ctrl/7(t)
  Local Ctrl/1(S_top) -> Mux/1
  Local Ctrl/2(S_bot) -> Mux/2
  Mux/1 -> g/1

== system MMC_Per_arm_outer_v5_G2_case2_clip_delay1p4_aligned/SM_u3 ==
  Local Ctrl : MATLAB Function  TreatAsAtomicUnit=on
  Mux : Mux  Inputs=2
  Neighbors : MATLAB Function  TreatAsAtomicUnit=on
  sm_id : Constant  Value=3
  g : Outport
  wires:
  [Vc_up] -> Neighbors/1(Vc_arm)
  sm_id/1 -> Neighbors/2(i), Local Ctrl/1(sm_id)
  [m_up] -> Local Ctrl/2(m_arm)
  [i_u] -> Local Ctrl/3(i_arm)
  Neighbors/1(Vc_i) -> Local Ctrl/4(Vc_i)
  Neighbors/2(Vc_prev) -> Local Ctrl/5(Vc_prev)
  Neighbors/3(Vc_next) -> Local Ctrl/6(Vc_next)
  [t] -> Local Ctrl/7(t)
  Local Ctrl/1(S_top) -> Mux/1
  Local Ctrl/2(S_bot) -> Mux/2
  Mux/1 -> g/1

== system MMC_Per_arm_outer_v5_G2_case2_clip_delay1p4_aligned/SM_u4 ==
  Local Ctrl : MATLAB Function  TreatAsAtomicUnit=on
  Mux : Mux  Inputs=2
  Neighbors : MATLAB Function  TreatAsAtomicUnit=on
  sm_id : Constant  Value=4
  g : Outport
  wires:
  [Vc_up] -> Neighbors/1(Vc_arm)
  sm_id/1 -> Neighbors/2(i), Local Ctrl/1(sm_id)
  [m_up] -> Local Ctrl/2(m_arm)
  [i_u] -> Local Ctrl/3(i_arm)
  Neighbors/1(Vc_i) -> Local Ctrl/4(Vc_i)
  Neighbors/2(Vc_prev) -> Local Ctrl/5(Vc_prev)
  Neighbors/3(Vc_next) -> Local Ctrl/6(Vc_next)
  [t] -> Local Ctrl/7(t)
  Local Ctrl/1(S_top) -> Mux/1
  Local Ctrl/2(S_bot) -> Mux/2
  Mux/1 -> g/1

== system MMC_Per_arm_outer_v5_G2_case2_clip_delay1p4_aligned/SM_u5 ==
  Local Ctrl : MATLAB Function  TreatAsAtomicUnit=on
  Mux : Mux  Inputs=2
  Neighbors : MATLAB Function  TreatAsAtomicUnit=on
  sm_id : Constant  Value=5
  g : Outport
  wires:
  [Vc_up] -> Neighbors/1(Vc_arm)
  sm_id/1 -> Neighbors/2(i), Local Ctrl/1(sm_id)
  [m_up] -> Local Ctrl/2(m_arm)
  [i_u] -> Local Ctrl/3(i_arm)
  Neighbors/1(Vc_i) -> Local Ctrl/4(Vc_i)
  Neighbors/2(Vc_prev) -> Local Ctrl/5(Vc_prev)
  Neighbors/3(Vc_next) -> Local Ctrl/6(Vc_next)
  [t] -> Local Ctrl/7(t)
  Local Ctrl/1(S_top) -> Mux/1
  Local Ctrl/2(S_bot) -> Mux/2
  Mux/1 -> g/1

== system MMC_Per_arm_outer_v5_G2_case2_clip_delay1p4_aligned/SM_u6 ==
  Local Ctrl : MATLAB Function  TreatAsAtomicUnit=on
  Mux : Mux  Inputs=2
  Neighbors : MATLAB Function  TreatAsAtomicUnit=on
  sm_id : Constant  Value=6
  g : Outport
  wires:
  [Vc_up] -> Neighbors/1(Vc_arm)
  sm_id/1 -> Neighbors/2(i), Local Ctrl/1(sm_id)
  [m_up] -> Local Ctrl/2(m_arm)
  [i_u] -> Local Ctrl/3(i_arm)
  Neighbors/1(Vc_i) -> Local Ctrl/4(Vc_i)
  Neighbors/2(Vc_prev) -> Local Ctrl/5(Vc_prev)
  Neighbors/3(Vc_next) -> Local Ctrl/6(Vc_next)
  [t] -> Local Ctrl/7(t)
  Local Ctrl/1(S_top) -> Mux/1
  Local Ctrl/2(S_bot) -> Mux/2
  Mux/1 -> g/1

== system MMC_Per_arm_outer_v5_G2_case2_clip_delay1p4_aligned/SM_u7 ==
  Local Ctrl : MATLAB Function  TreatAsAtomicUnit=on
  Mux : Mux  Inputs=2
  Neighbors : MATLAB Function  TreatAsAtomicUnit=on
  sm_id : Constant  Value=7
  g : Outport
  wires:
  [Vc_up] -> Neighbors/1(Vc_arm)
  sm_id/1 -> Neighbors/2(i), Local Ctrl/1(sm_id)
  [m_up] -> Local Ctrl/2(m_arm)
  [i_u] -> Local Ctrl/3(i_arm)
  Neighbors/1(Vc_i) -> Local Ctrl/4(Vc_i)
  Neighbors/2(Vc_prev) -> Local Ctrl/5(Vc_prev)
  Neighbors/3(Vc_next) -> Local Ctrl/6(Vc_next)
  [t] -> Local Ctrl/7(t)
  Local Ctrl/1(S_top) -> Mux/1
  Local Ctrl/2(S_bot) -> Mux/2
  Mux/1 -> g/1

== system MMC_Per_arm_outer_v5_G2_case2_clip_delay1p4_aligned/SM_u8 ==
  Local Ctrl : MATLAB Function  TreatAsAtomicUnit=on
  Mux : Mux  Inputs=2
  Neighbors : MATLAB Function  TreatAsAtomicUnit=on
  sm_id : Constant  Value=8
  g : Outport
  wires:
  [Vc_up] -> Neighbors/1(Vc_arm)
  sm_id/1 -> Neighbors/2(i), Local Ctrl/1(sm_id)
  [m_up] -> Local Ctrl/2(m_arm)
  [i_u] -> Local Ctrl/3(i_arm)
  Neighbors/1(Vc_i) -> Local Ctrl/4(Vc_i)
  Neighbors/2(Vc_prev) -> Local Ctrl/5(Vc_prev)
  Neighbors/3(Vc_next) -> Local Ctrl/6(Vc_next)
  [t] -> Local Ctrl/7(t)
  Local Ctrl/1(S_top) -> Mux/1
  Local Ctrl/2(S_bot) -> Mux/2
  Mux/1 -> g/1

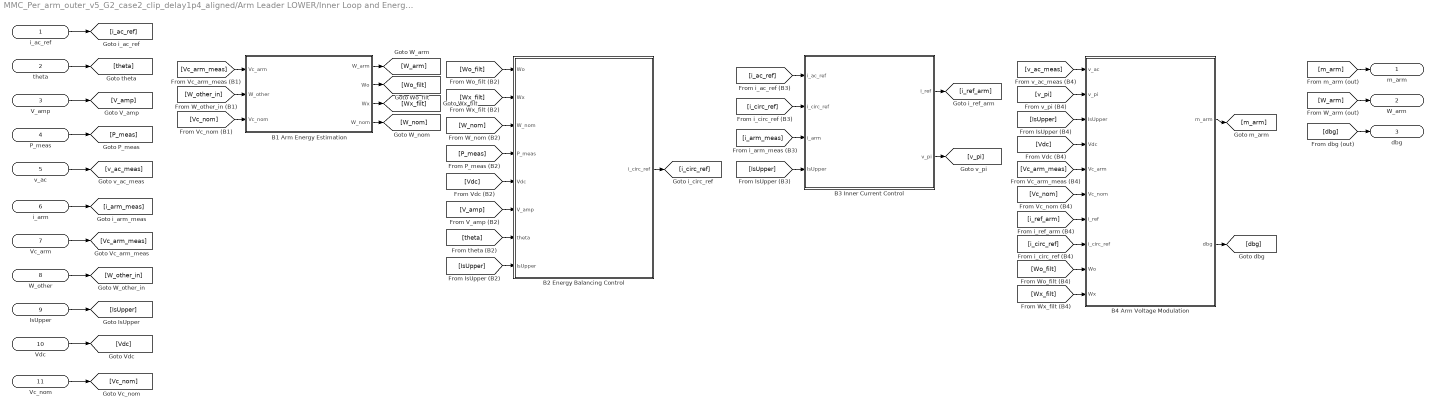
== system MMC_Per_arm_outer_v5_G2_case2_clip_delay1p4_aligned/Arm Leader LOWER/Inner Loop and Energy Balancing ==
  i_ac_ref : Inport
  theta : Inport  Port=2
  V_amp : Inport  Port=3
  P_meas : Inport  Port=4
  v_ac : Inport  Port=5
  i_arm : Inport  Port=6
  Vc_arm : Inport  Port=7
  W_other : Inport  Port=8
  IsUpper : Inport  Port=9
  Vdc : Inport  Port=10
  Vc_nom : Inport  Port=11
  B1 Arm Energy Estimation : MATLAB Function  TreatAsAtomicUnit=on
  B2 Energy Balancing Control : MATLAB Function  TreatAsAtomicUnit=on
  B3 Inner Current Control : MATLAB Function  TreatAsAtomicUnit=on
  B4 Arm Voltage Modulation : MATLAB Function  TreatAsAtomicUnit=on
  m_arm : Outport
  W_arm : Outport  Port=2
  dbg : Outport  Port=3
  wires:
  i_ac_ref/1 -> [i_ac_ref]
  theta/1 -> [theta]
  V_amp/1 -> [V_amp]
  P_meas/1 -> [P_meas]
  v_ac/1 -> [v_ac_meas]
  i_arm/1 -> [i_arm_meas]
  Vc_arm/1 -> [Vc_arm_meas]
  W_other/1 -> [W_other_in]
  IsUpper/1 -> [IsUpper]
  Vdc/1 -> [Vdc]
  Vc_nom/1 -> [Vc_nom]
  [Vc_arm_meas] -> B1 Arm Energy Estimation/1(Vc_arm)
  [W_other_in] -> B1 Arm Energy Estimation/2(W_other)
  [Vc_nom] -> B1 Arm Energy Estimation/3(Vc_nom)
  B1 Arm Energy Estimation/1(W_arm) -> [W_arm]
  B1 Arm Energy Estimation/2(Wo) -> [Wo_filt]
  B1 Arm Energy Estimation/3(Wx) -> [Wx_filt]
  B1 Arm Energy Estimation/4(W_nom) -> [W_nom]
  [Wo_filt] -> B2 Energy Balancing Control/1(Wo)
  [Wx_filt] -> B2 Energy Balancing Control/2(Wx)
  [W_nom] -> B2 Energy Balancing Control/3(W_nom)
  [P_meas] -> B2 Energy Balancing Control/4(P_meas)
  [Vdc] -> B2 Energy Balancing Control/5(Vdc)
  [V_amp] -> B2 Energy Balancing Control/6(V_amp)
  [theta] -> B2 Energy Balancing Control/7(theta)
  [IsUpper] -> B2 Energy Balancing Control/8(IsUpper)
  B2 Energy Balancing Control/1(i_circ_ref) -> [i_circ_ref]
  [i_ac_ref] -> B3 Inner Current Control/1(i_ac_ref)
  [i_circ_ref] -> B3 Inner Current Control/2(i_circ_ref)
  [i_arm_meas] -> B3 Inner Current Control/3(i_arm)
  [IsUpper] -> B3 Inner Current Control/4(IsUpper)
  B3 Inner Current Control/1(i_ref) -> [i_ref_arm]
  B3 Inner Current Control/2(v_pi) -> [v_pi]
  [v_ac_meas] -> B4 Arm Voltage Modulation/1(v_ac)
  [v_pi] -> B4 Arm Voltage Modulation/2(v_pi)
  [IsUpper] -> B4 Arm Voltage Modulation/3(IsUpper)
  [Vdc] -> B4 Arm Voltage Modulation/4(Vdc)
  [Vc_arm_meas] -> B4 Arm Voltage Modulation/5(Vc_arm)
  [Vc_nom] -> B4 Arm Voltage Modulation/6(Vc_nom)
  [i_ref_arm] -> B4 Arm Voltage Modulation/7(i_ref)
  [i_circ_ref] -> B4 Arm Voltage Modulation/8(i_circ_ref)
  [Wo_filt] -> B4 Arm Voltage Modulation/9(Wo)
  [Wx_filt] -> B4 Arm Voltage Modulation/10(Wx)
  B4 Arm Voltage Modulation/1(m_arm) -> [m_arm]
  B4 Arm Voltage Modulation/2(dbg) -> [dbg]
  [m_arm] -> m_arm/1
  [W_arm] -> W_arm/1
  [dbg] -> dbg/1

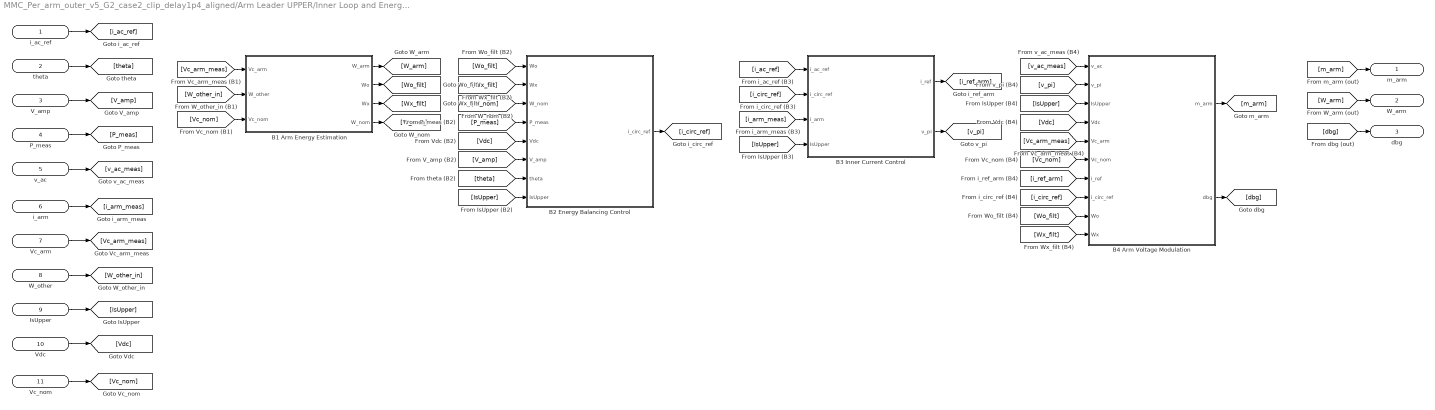
== system MMC_Per_arm_outer_v5_G2_case2_clip_delay1p4_aligned/Arm Leader UPPER/Inner Loop and Energy Balancing ==
  i_ac_ref : Inport
  theta : Inport  Port=2
  V_amp : Inport  Port=3
  P_meas : Inport  Port=4
  v_ac : Inport  Port=5
  i_arm : Inport  Port=6
  Vc_arm : Inport  Port=7
  W_other : Inport  Port=8
  IsUpper : Inport  Port=9
  Vdc : Inport  Port=10
  Vc_nom : Inport  Port=11
  B1 Arm Energy Estimation : MATLAB Function  TreatAsAtomicUnit=on
  B2 Energy Balancing Control : MATLAB Function  TreatAsAtomicUnit=on
  B3 Inner Current Control : MATLAB Function  TreatAsAtomicUnit=on
  B4 Arm Voltage Modulation : MATLAB Function  TreatAsAtomicUnit=on
  m_arm : Outport
  W_arm : Outport  Port=2
  dbg : Outport  Port=3
  wires:
  i_ac_ref/1 -> [i_ac_ref]
  theta/1 -> [theta]
  V_amp/1 -> [V_amp]
  P_meas/1 -> [P_meas]
  v_ac/1 -> [v_ac_meas]
  i_arm/1 -> [i_arm_meas]
  Vc_arm/1 -> [Vc_arm_meas]
  W_other/1 -> [W_other_in]
  IsUpper/1 -> [IsUpper]
  Vdc/1 -> [Vdc]
  Vc_nom/1 -> [Vc_nom]
  [Vc_arm_meas] -> B1 Arm Energy Estimation/1(Vc_arm)
  [W_other_in] -> B1 Arm Energy Estimation/2(W_other)
  [Vc_nom] -> B1 Arm Energy Estimation/3(Vc_nom)
  B1 Arm Energy Estimation/1(W_arm) -> [W_arm]
  B1 Arm Energy Estimation/2(Wo) -> [Wo_filt]
  B1 Arm Energy Estimation/3(Wx) -> [Wx_filt]
  B1 Arm Energy Estimation/4(W_nom) -> [W_nom]
  [Wo_filt] -> B2 Energy Balancing Control/1(Wo)
  [Wx_filt] -> B2 Energy Balancing Control/2(Wx)
  [W_nom] -> B2 Energy Balancing Control/3(W_nom)
  [P_meas] -> B2 Energy Balancing Control/4(P_meas)
  [Vdc] -> B2 Energy Balancing Control/5(Vdc)
  [V_amp] -> B2 Energy Balancing Control/6(V_amp)
  [theta] -> B2 Energy Balancing Control/7(theta)
  [IsUpper] -> B2 Energy Balancing Control/8(IsUpper)
  B2 Energy Balancing Control/1(i_circ_ref) -> [i_circ_ref]
  [i_ac_ref] -> B3 Inner Current Control/1(i_ac_ref)
  [i_circ_ref] -> B3 Inner Current Control/2(i_circ_ref)
  [i_arm_meas] -> B3 Inner Current Control/3(i_arm)
  [IsUpper] -> B3 Inner Current Control/4(IsUpper)
  B3 Inner Current Control/1(i_ref) -> [i_ref_arm]
  B3 Inner Current Control/2(v_pi) -> [v_pi]
  [v_ac_meas] -> B4 Arm Voltage Modulation/1(v_ac)
  [v_pi] -> B4 Arm Voltage Modulation/2(v_pi)
  [IsUpper] -> B4 Arm Voltage Modulation/3(IsUpper)
  [Vdc] -> B4 Arm Voltage Modulation/4(Vdc)
  [Vc_arm_meas] -> B4 Arm Voltage Modulation/5(Vc_arm)
  [Vc_nom] -> B4 Arm Voltage Modulation/6(Vc_nom)
  [i_ref_arm] -> B4 Arm Voltage Modulation/7(i_ref)
  [i_circ_ref] -> B4 Arm Voltage Modulation/8(i_circ_ref)
  [Wo_filt] -> B4 Arm Voltage Modulation/9(Wo)
  [Wx_filt] -> B4 Arm Voltage Modulation/10(Wx)
  B4 Arm Voltage Modulation/1(m_arm) -> [m_arm]
  B4 Arm Voltage Modulation/2(dbg) -> [dbg]
  [m_arm] -> m_arm/1
  [W_arm] -> W_arm/1
  [dbg] -> dbg/1

== matlab function MMC_Per_arm_outer_v5_G2_case2_clip_delay1p4_aligned/SM_u3/Neighbors ==
  data: Vc_arm input; Vc_i output; i input; Vc_prev output; Vc_next output
function [Vc_i, Vc_prev, Vc_next] = get_neighbors(Vc_arm, i)
%#codegen
% =========================================================================
% GET_NEIGHBORS  -  Ring-link emulation for submodule number i
% -------------------------------------------------------------------------
% Block     : "Neighbors" inside every SM_ux / SM_lx subsystem
% Rate      : Ts = 10 us
% Instances : 16 (one per submodule)
% Purpose   : in simulation the whole capacitor-voltage vector of the arm is
%             available, but a real submodule only knows its OWN voltage and
%             the voltages of its two ring neighbours. This block hides
%             everything else, so the local controller stays truly local.
% Inputs    : Vc_arm  N x 1 vector of capacitor voltages of the arm (V)
%             i       own submodule index, 1..N
% Outputs   : Vc_i    own capacitor voltage (V)
%             Vc_prev voltage of the previous ring neighbour (V)
%             Vc_next voltage of the next ring neighbour (V)
% =========================================================================

%% ---------------- PARAMETERS ----------------
N = 8;                                   % submodules per arm (= length of Vc_arm, the Mux of the 8 HB voltages)
ND = 140;                             % ALIGNED-DELAY case: own AND neighbour values delayed by ND samples (Ts = 10 us -> 1.4 ms)
persistent buf_i buf_p buf_n idx         % circular buffers of the own sample and the two neighbour links, and the index

%% ---------------- 1. own index, made safe ----------------
k = min(max(round(i), 1), N);            % round to an integer and clamp to [1, N] (protects against a bad sm_id)

%% ---------------- 2. own voltage ----------------
Vc_i = Vc_arm(k);                        % own capacitor voltage

%% ---------------- 3. ring neighbours (circular: SM1 and SMN are neighbours) ----------------
if k == 1                                % first submodule of the ring
    Vc_prev = Vc_arm(N);                 % previous neighbour wraps around to the last submodule
    Vc_next = Vc_arm(2);                 % next neighbour is SM2
elseif k == N                            % last submodule of the ring
    Vc_prev = Vc_arm(N - 1);             % previous neighbour is SM(N-1)
    Vc_next = Vc_arm(1);                 % next neighbour wraps around to SM1
else                                     % any submodule in the middle
    Vc_prev = Vc_arm(k - 1);             % previous neighbour
    Vc_next = Vc_arm(k + 1);             % next neighbour
end

%% ---------------- 4. time-aligned delay: own sample and neighbour links delayed by the same ND (ALIGNED-DELAY case) ----------------
if isempty(buf_i)                        % first call
    buf_i = Vc_i    * ones(ND, 1);       % buffers start filled with the first values: no false error during the first ND samples
    buf_p = Vc_prev * ones(ND, 1);
    buf_n = Vc_next * ones(ND, 1);
    idx   = 1;
end
d_i    = buf_i(idx);                     % own voltage ND samples ago (same instant as the neighbour values)
d_prev = buf_p(idx);                     % value sent by the previous neighbour ND samples ago
d_next = buf_n(idx);                     % value sent by the next neighbour ND samples ago
buf_i(idx) = Vc_i;                       % store the fresh values in the slot just read
buf_p(idx) = Vc_prev;
buf_n(idx) = Vc_next;
idx = idx + 1;                           % advance the circular index
if idx > ND
    idx = 1;
end
Vc_i    = d_i;                           % the local controller compares three values of the SAME instant t - tau
Vc_prev = d_prev;
Vc_next = d_next;
end
